simulink model "SMC_AEM_observador_atChatt"  (R2026b)
settings: Solver=VariableStepAuto  StopTime=30  FixedStep=1  RelTol=1e-5
settings Model: Creator=Yahoff  LastModifiedBy=nestorhernandezcastellanos

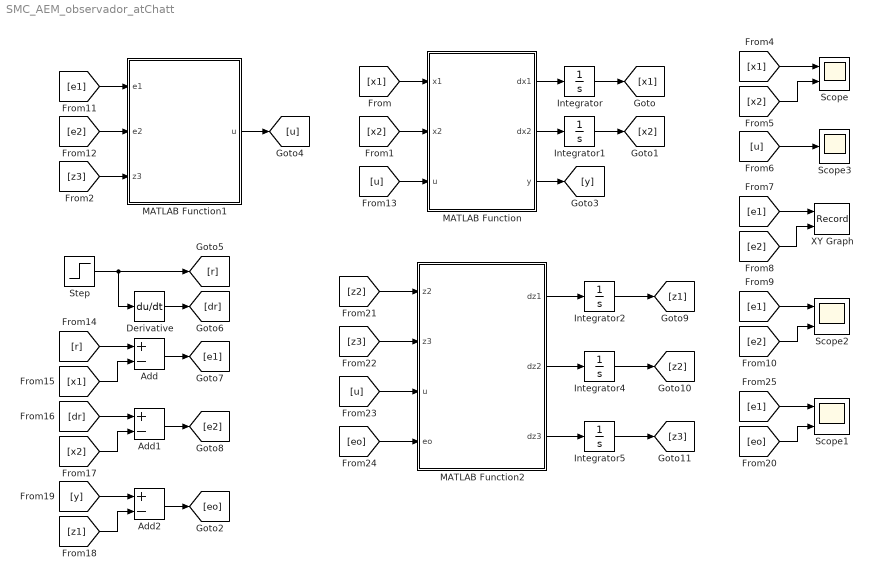
== system SMC_AEM_observador_atChatt ==
  Add : Sum  Inputs=+-
  Add1 : Sum  Inputs=+-
  Add2 : Sum  Inputs=+-
  Derivative : Derivative
  Integrator : Integrator  InitialCondition=2
  Integrator1 : Integrator  InitialCondition=-5
  Integrator2 : Integrator
  Integrator4 : Integrator
  Integrator5 : Integrator
  MATLAB Function : MATLAB Function  TreatAsAtomicUnit=on
  MATLAB Function1 : MATLAB Function  TreatAsAtomicUnit=on
  MATLAB Function2 : MATLAB Function  TreatAsAtomicUnit=on
  Scope : Scope  NumInputPorts=2
      settings: ActiveDisplayYMinimum=-3.7914093492139536  ActiveDisplayYMaximum=12.006885693769638
  Scope1 : Scope  NumInputPorts=2
      settings: ActiveDisplayYMinimum=-3.1027277880638686  ActiveDisplayYMaximum=5.89875712702713
  Scope2 : Scope  NumInputPorts=2
      settings: ActiveDisplayYMinimum=-0.57287009620433638  ActiveDisplayYMaximum=6.5079232278110926  DataLoggingVariableName=ScopeData2
  Scope3 : Scope
      settings: ActiveDisplayYMinimum=-5.7361371023584753E+6  ActiveDisplayYMaximum=2.0896222186681181E+6  DataLoggingVariableName=ScopeData3
  Step : Step  FinalValue=5  SampleTime=0
  XY Graph : Record  NumPorts=2.0  FileSettingsInternal="{\"entries\":[{\"content\":{\"excelSettings\":{\"content\":{},\"type\":\"Streamout.ExcelSettings\"},\"parquetSettings\":{\"content\":{},\"type\":\"Streamout.ParquetSettings\"}},\"type\":\"Streamout.FileSettingStorage\",\"uuid\":\"\"}],\"packageUris\":[\"http:\\/\\/schema.mathworks.com\\/mf0\\/streamout_blocks\\/R2020a\"],\"version\":\"1.0\"}"  FrameSettings=[0, 0]  Layout=[1 1]  SignalsInternal="{\"entries\":[{\"content\":{\"signals\":[{\"content\":{\"blockPath\":[],\"dimensions\":[1],\"domain\":\"\",\"lineColor\":\"#a2142f\",\"plots\":[ 1 ],\"port\":1,\"sid\":[\"\"],\"signalID\":1,\"signalName\":\"From7\"},\"type\":\"RecordBlkView.Signal\",\"uuid\":\"\"},{\"content\":{\"blockPath\":[],\"dimensions\":[1],\"domain\":\"\",\"lineColor\":\"#139fff\",\"plots\":[ 1 ],\"port\":2,\"sid\":[\"\"],\"signalID\":2,\"signalName\":\"From8\"},\"type\":\"RecordBlkView.Signal\",\"uuid\":\"\"}]},\"type\":\"RecordBlkView.InputSignals\",\"uuid\":\"\"}],\"packageUris\":[\"http:\\/\\/schema.mathworks.com\\/mf0\\/streamout_blocks\\/R2020a\"],\"version\":\"1.0\"}"  VisualizationBindings="{\"xyplotplugin\":{\"info\":[{\"series\":[{\"bindingParametersList\":[{\"parameter\":\"X-Axis\",\"signalID\":1,\"signalName\":\"From7\"},{\"parameter\":\"Y-Axis\",\"signalID\":2,\"signalName\":\"From8\"}],\"seriesID\":0}],\"subplotID\":1}]}}"  CompatibilityTag=XY
  wires:
  MATLAB Function/1(dx1) -> Integrator/1
  MATLAB Function/2(dx2) -> Integrator1/1
  Integrator/1 -> [x1]
  Integrator1/1 -> [x2]
  [x1] -> MATLAB Function/1(x1)
  [x2] -> MATLAB Function/2(x2)
  [z3] -> MATLAB Function1/3(z3)
  [x1] -> Scope/1
  [x2] -> Scope/2
  [u] -> Scope3/1
  [e1] -> XY Graph/1
  [e2] -> XY Graph/2
  [e1] -> Scope2/1
  [e2] -> Scope2/2
  MATLAB Function1/1(u) -> [u]
  Step/1 -> [r], Derivative/1
  Derivative/1 -> [dr]
  [e1] -> MATLAB Function1/1(e1)
  [e2] -> MATLAB Function1/2(e2)
  [u] -> MATLAB Function/3(u)
  [r] -> Add/1
  [x1] -> Add/2
  Add/1 -> [e1]
  Add1/1 -> [e2]
  [x2] -> Add1/2
  [dr] -> Add1/1
  MATLAB Function2/2(dz2) -> Integrator4/1
  MATLAB Function2/1(dz1) -> Integrator2/1
  MATLAB Function2/3(dz3) -> Integrator5/1
  Integrator5/1 -> [z3]
  Integrator2/1 -> [z1]
  Integrator4/1 -> [z2]
  [z3] -> MATLAB Function2/2(z3)
  [u] -> MATLAB Function2/3(u)
  [z2] -> MATLAB Function2/1(z2)
  [eo] -> MATLAB Function2/4(eo)
  Add2/1 -> [eo]
  [y] -> Add2/1
  [z1] -> Add2/2
  [eo] -> Scope1/2
  [e1] -> Scope1/1
  MATLAB Function/3(y) -> [y]

== matlab function SMC_AEM_observador_atChatt/MATLAB Function1 ==
  data: e1 input; u output; e2 input; z3 input
function u = controlador(e1,e2,z3)

m = 6;
K = 15;

% Superficie de deslizamiento
sigma = e2 + m*e1;

% Ley de control
u = z3 + m*e2 + K*sign(sigma);

== matlab function SMC_AEM_observador_atChatt/MATLAB Function ==
  data: x1 input; x2 input; u input; dx1 output; dx2 output; y output
function [dx1,dx2, y] = planta(x1,x2,u)

dx1 = sin(x1+x2) + x2;
dx2 = cos(x1+x2) + u;

y = x1;

== matlab function SMC_AEM_observador_atChatt/MATLAB Function2 ==
  data: z2 input; z3 input; u input; dz1 output; eo input; dz2 output; dz3 output
function [dz1, dz2, dz3] = LESO(z2, z3, u, eo)

b=1;

Ko1 = 45.9089;
Ko2 = 1156.247;
Ko3 = 8654.473;

% Observador
dz1 = z2 + Ko1*eo;
dz2 = z3 + b*u + Ko2*eo;
dz3 = Ko3*eo;
